simulink model "Maxom_fcs_noncascaded"  (R2025b)
settings: Solver=ode45  StartTime=0.0  StopTime=0.30  FixedStep=1e-6  MaxStep=1e-5  RelTol=1e-4  EnableMultiTasking=on
values from neighbouring files (symbols this model uses):
  Bfric = 0    [PMSMpara.m]
  ffai = 0.008667    [PMSMpara.m]
  Imax = 20    [PMSMpara.m]
  J = 0.044e-4    (= 4.4e-06)    [PMSMpara.m]
  kis = 0    [PMSMpara.m]
  kps = fsc*6.28*J/Kt    (= 0.364364007978)    [PMSMpara.m]
  Kt = np*1.5*ffai    (= 0.0910035)    [PMSMpara.m]
  Ld = Ls    (= 0.00045)    [PMSMpara.m]
  Lq = Ls    (= 0.00045)    [PMSMpara.m]
  np = 7    [PMSMpara.m]
  Rs = 0.5    [PMSMpara.m]
  Tcur = 1/32000    (= 3.125e-05)    [PMSMpara.m]
  Tpwm = 1/32000    (= 3.125e-05)    [PMSMpara.m]
  Tspd = 1/32000    (= 3.125e-05)    [PMSMpara.m]
  wn = 311040    [PMSMpara.m]
  zeta = 1    [PMSMpara.m]
undefined symbols (not defined in the file or in its folder): dspblkCoreblockFVToolHelper, gcbh
libraries: simulink x4, slpidlib x2, spsUniversalBridgeLib x1, spsCurrentMeasurementLib x1, EasyGo_Machine_lib x1, spsPermanentMagnetSynchronousMachineLib x1, spsSVPWMGenerator2LevelLib x1, spsDCVoltageSourceLib x1, sps_lib x1
(part 4 of 4)

== matlab function Maxom_fcs_noncascaded/f_pmsm_foc_sl/MATLAB Function4 ==
  data: i_pred output; ia input; gg output; ib input; ic input; id_ref input; we_ref input; we input; theta_mech input; Vdc input; Ld input; Lq input; Rs input; lambda_f input; Tcur input; lambda_c input; Kp_we input; Ki_we input; Kaw input; iq_max input
function [i_pred, gg] = fcs_smdo_1s_we_no_torque( ...
    ia, ib, ic, id_ref, we_ref, we, theta_mech, Vdc, Ld, Lq, Rs, ...
    lambda_f, Tcur, lambda_c, Kp_we, Ki_we, Kaw, iq_max)
%#codegen
% Electrical-speed PI produces iq_ref internally.
% we and we_ref must both be electrical angular speed [rad/s].

np = single(7);

ia = single(ia); ib = single(ib); ic = single(ic);
id_ref = single(id_ref);
we_ref = single(we_ref); we = single(we);
theta_e = single(mod(np*single(theta_mech) - single(pi/2), single(2*pi)));
Ts = single(Tcur);

Vdc = single(Vdc); Ld = single(Ld); Lq = single(Lq); Rs = single(Rs);
lambda_f = single(lambda_f); lambda_c = single(lambda_c);
Kp_we = single(Kp_we); Ki_we = single(Ki_we);
Kaw = single(Kaw); iq_max = single(iq_max);

inv_Ld = single(1)/Ld;
inv_Lq = single(1)/Lq;
TsLd = Ts*inv_Ld;
TsLq = Ts*inv_Lq;

ct = single(cos(theta_e));
st = single(sin(theta_e));
sqrt3 = single(sqrt(3));

i_alpha = single(2/3)*(ia - single(0.5)*ib - single(0.5)*ic);
i_beta  = single(2/3)*(sqrt3/single(2))*(ib - ic);
is_d = single( ct*i_alpha + st*i_beta);
is_q = single(-st*i_alpha + ct*i_beta);
x_k  = single([is_d; is_q]);

AB = single(0.6); BB = single(1.2);
K1 = single(6000); K2 = single(6000);
K3 = single(2.5e5); K4 = single(1e6);

V = single([0 0 0; 1 0 0; 1 1 0; 0 1 0; ...
            0 1 1; 0 0 1; 1 0 1; 1 1 1]);
Kcl = single(2/3)*Vdc*single([1 -0.5 -0.5; ...
                              0 sqrt(3)/2 -sqrt(3)/2]);

persistent z1 z2 s_prev Ispd
if isempty(z1)
    z1 = x_k;
    z2 = zeros(2,1,'single');
    s_prev = zeros(3,1,'single');
    Ispd = single(0);
end

% ===================== SPEED PI: NO TORQUE FEED-FORWARD ==================
e_we = we_ref - we;
iq_unsat = Kp_we*e_we + Ispd;
iq_ref = max(min(iq_unsat, iq_max), -iq_max);

% Back-calculation anti-windup. Ispd is the integral contribution in amperes.
Ispd = Ispd + Ts*(Ki_we*e_we + Kaw*(iq_ref - iq_unsat));

% ===================== SMDO UPDATE =======================================
% theta_e(k-1) approximately equals theta_e(k) - we(k)*Ts.
th_p = theta_e - we*Ts;
ctp = single(cos(th_p));
stp = single(sin(th_p));
v_app = single([ctp stp; -stp ctp])*(Kcl*s_prev);

e = z1 - x_k;
ae = abs(e); se = sign(e);
sa1 = ae.^AB .* se;
sb1 = ae.^BB .* se;
sa2 = ae.^(single(2)*AB-single(1)) .* se;
sb2 = ae.^(single(2)*BB-single(1)) .* se;

f_nom = single([(-Rs*x_k(1) + we*Lq*x_k(2))*inv_Ld; ...
                (-Rs*x_k(2) - we*Ld*x_k(1) - we*lambda_f)*inv_Lq]);
g_u = single([v_app(1)*inv_Ld; v_app(2)*inv_Lq]);

z1 = z1 + Ts*(f_nom + g_u + z2 - K1*sa1 - K2*sb1);
z2 = z2 + Ts*(-K3*sa2 - K4*sb2);
d_hat = z2;

% ===================== ALL 8 dq VOLTAGES ================================
Vab = Kcl*V';
Vdq = single([ct st; -st ct])*Vab;

% ===================== CURRENT PREDICTION BASE ===========================
id_base = is_d + TsLd*(-Rs*is_d + we*Lq*is_q) ...
          + Ts*d_hat(1);
iq_base = is_q + TsLq*(-Rs*is_q - we*Ld*is_d - we*lambda_f) ...
          + Ts*d_hat(2);

% ===================== SINGLE-STEP FCS SEARCH ============================
g_best = single(9e20);
idx = int32(1);
id_best = single(0);
iq_best = single(0);

for n = 1:8
    id_p = id_base + TsLd*Vdq(1,n);
    iq_p = iq_base + TsLq*Vdq(2,n);

    ed = id_ref - id_p;
    eq = iq_ref - iq_p;
    g = ed*ed + lambda_c*(eq*eq);

    if g < g_best
        g_best = g;
        idx = int32(n);
        id_best = id_p;
        iq_best = iq_p;
    end
end

s_prev = V(idx,:)';
Sa = s_prev(1); Sb = s_prev(2); Sc = s_prev(3);

gg = single([Sa; 1-Sa; Sb; 1-Sb; Sc; 1-Sc]);
i_pred = single([id_best, iq_best]);
end
